simulink model "drive_gearbox"  (R2026b)
settings: Solver=VariableStepAuto
undefined symbols (not defined in the file or in its folder): P
libraries: fl_lib x13, nesl_utility x3
settings Model: Creator=aomar  LastModifiedBy=aomar

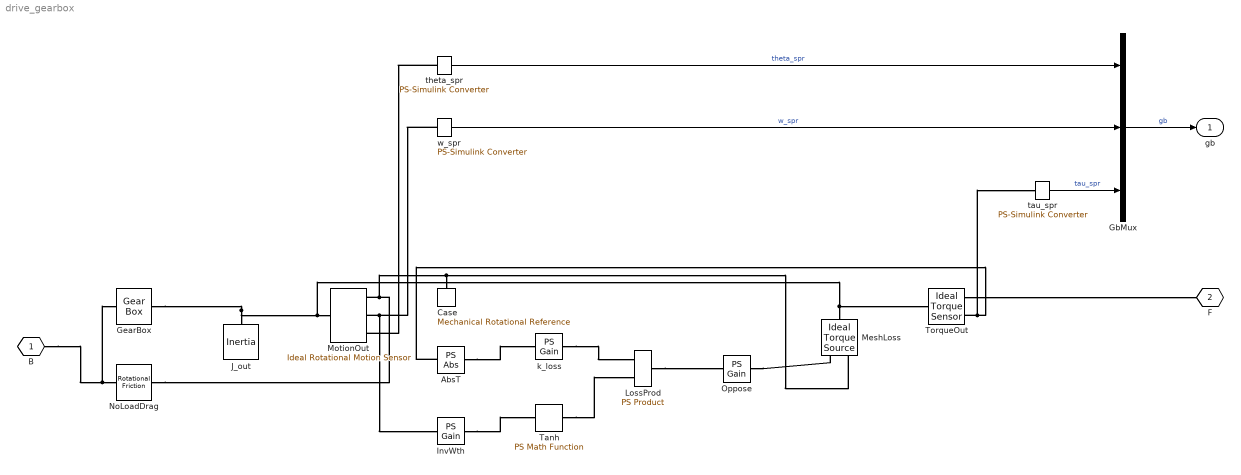
== system drive_gearbox ==
  AbsT : fl_lib/Physical Signals/Nonlinear Operators/PS Abs  ZeroCross=true
  Case : fl_lib/Mechanical/Rotational Elements/Mechanical Rotational Reference
  GbMux : Mux  Inputs=3
  GearBox : fl_lib/Mechanical/Mechanisms/Gear Box  ratio=P.drive.gear.N  t_in_specify=off  t_in_priority=None  t_in=0 N*m  t_in_nominal_specify=off  t_in_nominal_value=1  t_in_nominal_unit=N*m  t_out_specify=off  t_out_priority=None  t_out=0 N*m  t_out_nominal_specify=off  t_out_nominal_value=1  t_out_nominal_unit=N*m
  InvWth : fl_lib/Physical Signals/Functions/PS Gain  gain=1/P.drive.gear.w_th s/rad
  J_out : fl_lib/Mechanical/Rotational Elements/Inertia  inertia=P.drive.gear.J_out kg*m^2  num_ports=foundation.enum.numPorts2.one  w_specify=off  w_priority=High  w=0 rad/s  w_nominal_specify=off  w_nominal_value=1  w_nominal_unit=rad/s  t_specify=off  t_priority=None  t=0 N*m  t_nominal_specify=off  t_nominal_value=1  t_nominal_unit=N*m
  LossProd : fl_lib/Physical Signals/Functions/PS Product
  MeshLoss : fl_lib/Mechanical/Mechanical Sources/Ideal Torque Source
  MotionOut : fl_lib/Mechanical/Mechanical Sensors/Ideal Rotational Motion Sensor  reference=foundation.enum.MeasurementReference.difference  acceleration_port=false  velocity_port=true  position_port=true  wrap_angle=false  offset=0 rad
  NoLoadDrag : fl_lib/Mechanical/Rotational Elements/Rotational Friction  brkwy_trq=P.drive.gear.T_nl_brk N*m  brkwy_vel=P.drive.gear.w_nl_brk rad/s  Col_trq=P.drive.gear.T_nl_C N*m  visc_coef=P.drive.gear.c_nl N*m*s/rad  w_specify=off  w_priority=None  w=0 rad/s  w_nominal_specify=off  w_nominal_value=1  w_nominal_unit=rad/s  t_specify=off  t_priority=None  t=0 N*m  t_nominal_specify=off  t_nominal_value=1  t_nominal_unit=N*m
  Oppose : fl_lib/Physical Signals/Functions/PS Gain  gain=-1
  Tanh : fl_lib/Physical Signals/Functions/PS Math Function  fcn_choice=foundation.enum.math_function.tanh  v=1
  TorqueOut : fl_lib/Mechanical/Mechanical Sensors/Ideal Torque Sensor
  k_loss : fl_lib/Physical Signals/Functions/PS Gain  gain=P.drive.gear.k_loss
  tau_spr : nesl_utility/PS-Simulink Converter  PhysicalDomain=network_engine_domain  SubClassName=ps_output  LeftPortType=input  RightPortType=output  PseudoPeriodic=off  Frequencies=[]  VectorFormat=inherit  Unit=N*m  AffineConversion=off
  theta_spr : nesl_utility/PS-Simulink Converter  PhysicalDomain=network_engine_domain  SubClassName=ps_output  LeftPortType=input  RightPortType=output  PseudoPeriodic=off  Frequencies=[]  VectorFormat=inherit  Unit=rad  AffineConversion=off
  w_spr : nesl_utility/PS-Simulink Converter  PhysicalDomain=network_engine_domain  SubClassName=ps_output  LeftPortType=input  RightPortType=output  PseudoPeriodic=off  Frequencies=[]  VectorFormat=inherit  Unit=rad/s  AffineConversion=off
  B : PMIOPort  Side=Left  ConnectionType=Connection: foundation.mechanical.rotational.rotational
  F : PMIOPort  Port=2  Side=Right  ConnectionType=Connection: foundation.mechanical.rotational.rotational
  gb : Outport  OutDataTypeStr=double
  wires:
  theta_spr/1 -> GbMux/1  "theta_spr"
  w_spr/1 -> GbMux/2  "w_spr"
  tau_spr/1 -> GbMux/3  "tau_spr"
  GbMux/1 -> gb/1  "gb"
  connections:
  TorqueOut/RConn2 -- AbsT/LConn1 -- tau_spr/LConn1
  AbsT/RConn1 -- k_loss/LConn1
  NoLoadDrag/LConn1 -- B/RConn1 -- GearBox/LConn1
  TorqueOut/RConn1 -- F/RConn1
  J_out/LConn1 -- GearBox/RConn1 -- MotionOut/LConn1 -- MeshLoss/LConn1 -- TorqueOut/LConn1
  InvWth/RConn1 -- Tanh/LConn1
  k_loss/RConn1 -- LossProd/LConn1
  Tanh/RConn1 -- LossProd/LConn2
  LossProd/RConn1 -- Oppose/LConn1
  Oppose/RConn1 -- MeshLoss/RConn1
  theta_spr/LConn1 -- MotionOut/RConn3
  MotionOut/RConn1 -- NoLoadDrag/RConn1 -- Case/LConn1 -- MeshLoss/RConn2
  MotionOut/RConn2 -- w_spr/LConn1 -- InvWth/LConn1
